simulink model "s_b4a4x32kf"  (R2018a)
settings: Solver=VariableStepDiscrete  StartTime=0.0  StopTime=1  RelTol=1e-3
undefined symbols (not defined in the file): fft_stages, n_bits_ants, n_bits_xengs
libraries: xbsIndex_r4 x22056, xbsReplacements_r4 x30, casper_library_misc x29, casper_library_scopes x15, xps_library x4
(part 125 of 227)

== system s_b4a4x32kf/sys0/xeng/auto_tap/dual_pol_cmac ==
  a1 : Inport
  a2 : Inport  Port=2
  acc_in : Inport  Port=3
  sync : Inport  Port=4
  valid_in : Inport  Port=5
  Concat : xbsIndex_r4/Concat  num_inputs=4  dbl_ovrd=off  block_type=concat
      settings: block_version=9.2.01
  Constant1 : xbsIndex_r4/Constant  const=0  gui_display_data_type=Fixed-point  arith_type=Unsigned  n_bits=1  bin_pt=0  preci_type=Single  exp_width=8  frac_width=24  explicit_period=on  period=1  equ=P=C  opselect=C  inp2=PCIN>>17  opr=+  inp1=P  carry=CIN  dbl_ovrd=off  block_type=constant
      settings: block_version=9.2.01
  Constant2 : xbsIndex_r4/Constant  const=0  gui_display_data_type=Fixed-point  arith_type=Unsigned  n_bits=1  bin_pt=0  preci_type=Single  exp_width=8  frac_width=24  explicit_period=on  period=1  equ=P=C  opselect=C  inp2=PCIN>>17  opr=+  inp1=P  carry=CIN  dbl_ovrd=off  block_type=constant
      settings: block_version=9.2.01
  Constant4 : xbsIndex_r4/Constant  const=0  gui_display_data_type=Fixed-point  arith_type=Unsigned  n_bits=1  bin_pt=0  preci_type=Single  exp_width=8  frac_width=24  explicit_period=on  period=1  equ=P=C  opselect=C  inp2=PCIN>>17  opr=+  inp1=P  carry=CIN  dbl_ovrd=off  block_type=constant
      settings: block_version=9.2.01
  Slice{,1,6,10} (4 alike) : xbsIndex_r4/Slice  nbits=2*n_bits  boolean_output=off  mode=Upper Bit Location + Width  bit1=0  base1=MSB of Input  bit0=0  base0=LSB of Input  dbl_ovrd=off  block_type=slice
      Slice settings: infoedit="Extracts a given range of bits from each input sample and presents it at the output.  The output type is ordinarily unsigned with binary point at zero, but can be Boolean when the slice is one bit wide.<P><P>Hardware notes: In hardware this block costs nothing."  block_version=9.2.01
      Slice1 settings: infoedit="Extracts a given range of bits from each input sample and presents it at the output.  The output type is ordinarily unsigned with binary point at zero, but can be Boolean when the slice is one bit wide.<P><P>Hardware notes: In hardware this block costs nothing."  block_version=9.2.01
      Slice10 settings: block_version=9.2.01
      Slice6 settings: infoedit="Extracts a given range of bits from each input sample and presents it at the output.  The output type is ordinarily unsigned with binary point at zero, but can be Boolean when the slice is one bit wide.<P><P>Hardware notes: In hardware this block costs nothing."  block_version=9.2.01
  Slice11 : xbsIndex_r4/Slice  nbits=2*n_bits_out  boolean_output=off  mode=Upper Bit Location + Width  bit1=-6*n_bits_out  base1=MSB of Input  bit0=0  base0=LSB of Input  dbl_ovrd=off  block_type=slice
      settings: infoedit="Extracts a given range of bits from each input sample and presents it at the output.  The output type is ordinarily unsigned with binary point at zero, but can be Boolean when the slice is one bit wide.<P><P>Hardware notes: In hardware this block costs nothing."  block_version=9.2.01
  Slice2 : xbsIndex_r4/Slice  nbits=2*n_bits_out  boolean_output=off  mode=Upper Bit Location + Width  bit1=0  base1=MSB of Input  bit0=0  base0=LSB of Input  dbl_ovrd=off  block_type=slice
      settings: infoedit="Extracts a given range of bits from each input sample and presents it at the output.  The output type is ordinarily unsigned with binary point at zero, but can be Boolean when the slice is one bit wide.<P><P>Hardware notes: In hardware this block costs nothing."  block_version=9.2.01
  Slice{3..4,7,9} (4 alike) : xbsIndex_r4/Slice  nbits=2*n_bits  boolean_output=off  mode=Upper Bit Location + Width  bit1=-2*n_bits  base1=MSB of Input  bit0=0  base0=LSB of Input  dbl_ovrd=off  block_type=slice
      Slice3 settings: infoedit="Extracts a given range of bits from each input sample and presents it at the output.  The output type is ordinarily unsigned with binary point at zero, but can be Boolean when the slice is one bit wide.<P><P>Hardware notes: In hardware this block costs nothing."  block_version=9.2.01
      Slice4 settings: infoedit="Extracts a given range of bits from each input sample and presents it at the output.  The output type is ordinarily unsigned with binary point at zero, but can be Boolean when the slice is one bit wide.<P><P>Hardware notes: In hardware this block costs nothing."  block_version=9.2.01
      Slice7 settings: infoedit="Extracts a given range of bits from each input sample and presents it at the output.  The output type is ordinarily unsigned with binary point at zero, but can be Boolean when the slice is one bit wide.<P><P>Hardware notes: In hardware this block costs nothing."  block_version=9.2.01
      Slice9 settings: block_version=9.2.01
  Slice5 : xbsIndex_r4/Slice  nbits=2*n_bits_out  boolean_output=off  mode=Upper Bit Location + Width  bit1=-2*n_bits_out  base1=MSB of Input  bit0=0  base0=LSB of Input  dbl_ovrd=off  block_type=slice
      settings: infoedit="Extracts a given range of bits from each input sample and presents it at the output.  The output type is ordinarily unsigned with binary point at zero, but can be Boolean when the slice is one bit wide.<P><P>Hardware notes: In hardware this block costs nothing."  block_version=9.2.01
  Slice8 : xbsIndex_r4/Slice  nbits=2*n_bits_out  boolean_output=off  mode=Upper Bit Location + Width  bit1=-4*n_bits_out  base1=MSB of Input  bit0=0  base0=LSB of Input  dbl_ovrd=off  block_type=slice
      settings: infoedit="Extracts a given range of bits from each input sample and presents it at the output.  The output type is ordinarily unsigned with binary point at zero, but can be Boolean when the slice is one bit wide.<P><P>Hardware notes: In hardware this block costs nothing."  block_version=9.2.01
  Terminator : Terminator
  Terminator1 : Terminator
  Terminator2 : Terminator
  cmac1 : Subsystem  Tag=cmac_delinked  mask(cmac){acc_len=256, n_bits_a=8, bin_pt_a=7, n_bits_b=8, bin_pt_b=7, quantization=Truncate, overflow=Wrap, mult_latency=4, add_latency=3, in_latency=0, conv_latency=0, multiplier_implementation=embedded multiplier core}
      mask prompts: acc_len "Number of Accumulations"; n_bits_a "Number of bits 'a'"; bin_pt_a "Binary point 'a'"; n_bits_b "Number of bits 'b'"; bin_pt_b "Binary point 'b'"; quantization "Quantisation"; mult_latency "Multiplier Latency"; add_latency "Adder Latency"; in_latency "Input Latency"; conv_latency "Convert Latency"; multiplier_implementation "Multiplier Implementation"
      mask help: A complex multiply-accumulate block. Full precision.
      mask init:
      | bit_growth = ceil(log2(acc_len));
      | n_bits_out = (n_bits_a + n_bits_b + 1 + bit_growth);
      | bin_pt_out=(bin_pt_a + bin_pt_b);
      | set_param(gcb,'LinkStatus','inactive');
      | set_param([gcb,'/cmult*'],'LinkStatus','inactive');
      | set_param([gcb,'/cmult*'],'multiplier_implementation',num2str(multiplier_implementation));
      | set_param([gcb,'/cmult*'],'mult_latency',num2str(mult_latency));
      | set_param([gcb,'/cmult*'],'conjugated','on');
      | set_param([gcb,'/cmult*'],'add_latency',num2str(add_latency));
      | set_param([gcb,'/cmult*'],'n_bits_ab',num2str(n_bits_out));
      | set_param([gcb,'/cmult*'],'n_bits_a',num2str(n_bits_a));
      | set_param([gcb,'/cmult*'],'n_bits_b',num2str(n_bits_b));
      | set_param([gcb,'/cmult*'],'bin_pt_a',num2str(bin_pt_a));
      | set_param([gcb,'/cmult*'],'bin_pt_b',num2str(bin_pt_b));
      | set_param([gcb,'/cmult*'],'bin_pt_ab',num2str(bin_pt_out));
      mask TypeOptions quantization: Truncate | Round  (unbiased: +/- Inf) | Round  (unbiased: Even Values)
      mask TypeOptions overflow: Wrap | Saturate | Flag as error
      mask TypeOptions multiplier_implementation: behavioral HDL | standard core | embedded multiplier core
  cmac2 : Subsystem  Tag=cmac_delinked  mask(cmac){acc_len=256, n_bits_a=8, bin_pt_a=7, n_bits_b=8, bin_pt_b=7, quantization=Truncate, overflow=Wrap, mult_latency=4, add_latency=3, in_latency=0, conv_latency=0, multiplier_implementation=embedded multiplier core}
      mask prompts: acc_len "Number of Accumulations"; n_bits_a "Number of bits 'a'"; bin_pt_a "Binary point 'a'"; n_bits_b "Number of bits 'b'"; bin_pt_b "Binary point 'b'"; quantization "Quantisation"; mult_latency "Multiplier Latency"; add_latency "Adder Latency"; in_latency "Input Latency"; conv_latency "Convert Latency"; multiplier_implementation "Multiplier Implementation"
      mask help: A complex multiply-accumulate block. Full precision.
      mask init: same as s_b4a4x32kf/sys0/xeng/auto_tap/dual_pol_cmac/cmac1
      mask TypeOptions quantization: Truncate | Round  (unbiased: +/- Inf) | Round  (unbiased: Even Values)
      mask TypeOptions overflow: Wrap | Saturate | Flag as error
      mask TypeOptions multiplier_implementation: behavioral HDL | standard core | embedded multiplier core
  cmac3 : Subsystem  Tag=cmac_delinked  mask(cmac){acc_len=256, n_bits_a=8, bin_pt_a=7, n_bits_b=8, bin_pt_b=7, quantization=Truncate, overflow=Wrap, mult_latency=4, add_latency=3, in_latency=0, conv_latency=0, multiplier_implementation=embedded multiplier core}
      mask prompts: acc_len "Number of Accumulations"; n_bits_a "Number of bits 'a'"; bin_pt_a "Binary point 'a'"; n_bits_b "Number of bits 'b'"; bin_pt_b "Binary point 'b'"; quantization "Quantisation"; mult_latency "Multiplier Latency"; add_latency "Adder Latency"; in_latency "Input Latency"; conv_latency "Convert Latency"; multiplier_implementation "Multiplier Implementation"
      mask help: A complex multiply-accumulate block. Full precision.
      mask init: same as s_b4a4x32kf/sys0/xeng/auto_tap/dual_pol_cmac/cmac1
      mask TypeOptions quantization: Truncate | Round  (unbiased: +/- Inf) | Round  (unbiased: Even Values)
      mask TypeOptions overflow: Wrap | Saturate | Flag as error
      mask TypeOptions multiplier_implementation: behavioral HDL | standard core | embedded multiplier core
  cmac4 : Subsystem  Tag=cmac_delinked  mask(cmac){acc_len=256, n_bits_a=8, bin_pt_a=7, n_bits_b=8, bin_pt_b=7, quantization=Truncate, overflow=Wrap, mult_latency=4, add_latency=3, in_latency=0, conv_latency=0, multiplier_implementation=embedded multiplier core}
      mask prompts: acc_len "Number of Accumulations"; n_bits_a "Number of bits 'a'"; bin_pt_a "Binary point 'a'"; n_bits_b "Number of bits 'b'"; bin_pt_b "Binary point 'b'"; quantization "Quantisation"; mult_latency "Multiplier Latency"; add_latency "Adder Latency"; in_latency "Input Latency"; conv_latency "Convert Latency"; multiplier_implementation "Multiplier Implementation"
      mask help: A complex multiply-accumulate block. Full precision.
      mask init: same as s_b4a4x32kf/sys0/xeng/auto_tap/dual_pol_cmac/cmac1
      mask TypeOptions quantization: Truncate | Round  (unbiased: +/- Inf) | Round  (unbiased: Even Values)
      mask TypeOptions overflow: Wrap | Saturate | Flag as error
      mask TypeOptions multiplier_implementation: behavioral HDL | standard core | embedded multiplier core
  acc_out : Outport
  valid_out : Outport  Port=2
  wires:
  acc_in/1 -> Slice2/1, Slice5/1, Slice8/1, Slice11/1
  a2/1 -> Slice10/1, Slice7/1, Slice4/1, Slice1/1
  a1/1 -> Slice9/1, Slice6/1, Slice3/1, Slice/1
  cmac4/1(acc_out) -> Concat/4
  cmac3/1(acc_out) -> Concat/3
  cmac2/1(acc_out) -> Concat/2
  cmac1/1(acc_out) -> Concat/1
  cmac4/2(valid_out) -> valid_out/1
  cmac3/2(valid_out) -> Terminator2/1
  cmac2/2(valid_out) -> Terminator1/1
  sync/1 -> cmac4/4(sync), cmac3/4(sync), cmac2/4(sync), cmac1/4(sync)
  Slice11/1 -> cmac4/3(acc_in)
  Slice10/1 -> cmac4/2(c+di)
  Slice9/1 -> cmac4/1(a+bi)
  Constant4/1 -> cmac3/5(valid_in)
  Slice8/1 -> cmac3/3(acc_in)
  Slice7/1 -> cmac3/2(c+di)
  Slice6/1 -> cmac3/1(a+bi)
  Constant1/1 -> cmac2/5(valid_in)
  cmac1/2(valid_out) -> Terminator/1
  valid_in/1 -> cmac4/5(valid_in)
  Concat/1 -> acc_out/1
  Slice5/1 -> cmac2/3(acc_in)
  Slice4/1 -> cmac2/2(c+di)
  Slice3/1 -> cmac2/1(a+bi)
  Slice2/1 -> cmac1/3(acc_in)
  Slice1/1 -> cmac1/2(c+di)
  Slice/1 -> cmac1/1(a+bi)
  Constant2/1 -> cmac1/5(valid_in)

== system s_b4a4x32kf/sys0/xeng/auto_tap/sync_delay ==
  In : Inport
  Constant : xbsIndex_r4/Constant  const=1  gui_display_data_type=Fixed-point  arith_type=Unsigned  n_bits=BitWidth  bin_pt=0  preci_type=Single  exp_width=8  frac_width=24  explicit_period=on  period=1  equ=P=C  opselect=C  inp2=PCIN>>17  opr=+  inp1=P  carry=CIN  dbl_ovrd=off  block_type=constant
      settings: block_version=9.1.01
  Constant1 : xbsIndex_r4/Constant  const=0  gui_display_data_type=Fixed-point  arith_type=Unsigned  n_bits=BitWidth  bin_pt=0  preci_type=Single  exp_width=8  frac_width=24  explicit_period=on  period=1  equ=P=C  opselect=C  inp2=PCIN>>17  opr=+  inp1=P  carry=CIN  dbl_ovrd=off  block_type=constant
      settings: block_version=9.1.01
  Constant2 : xbsIndex_r4/Constant  const=DelayLen  gui_display_data_type=Fixed-point  arith_type=Unsigned  n_bits=BitWidth  bin_pt=0  preci_type=Single  exp_width=8  frac_width=24  explicit_period=on  period=1  equ=P=C  opselect=C  inp2=PCIN>>17  opr=+  inp1=P  carry=CIN  dbl_ovrd=off  block_type=constant
      settings: block_version=9.1.01
  Constant3 : xbsIndex_r4/Constant  const=UseCounter  gui_display_data_type=Fixed-point  arith_type=Unsigned  n_bits=1  bin_pt=0  preci_type=Single  exp_width=8  frac_width=24  explicit_period=on  period=1  equ=P=C  opselect=C  inp2=PCIN>>17  opr=+  inp1=P  carry=CIN  dbl_ovrd=off  block_type=constant
      settings: block_version=9.1.01
  Counter : xbsIndex_r4/Counter  cnt_type=Free Running  cnt_to=Inf  operation=Down  start_count=0  cnt_by_val=1  arith_type=Unsigned  n_bits=BitWidth  bin_pt=0  load_pin=on  rst=off  en=on  explicit_period=on  period=1  use_behavioral_HDL=off  implementation=Fabric  use_rpm=on  dbl_ovrd=off  block_type=counter
      settings: xl_area=[0, 0, 0, 0, 0, 0, 0]  block_version=9.1.01
  Logical : xbsIndex_r4/Logical  logical_function=OR  inputs=2  en=off  latency=0  precision=Full  arith_type=Unsigned  n_bits=8  bin_pt=2  align_bp=on  dbl_ovrd=off  block_type=logical
      settings: xl_area=[0, 0, 0, 0, 0, 0, 0]  block_version=9.1.01
  Mux : xbsIndex_r4/Mux  inputs=2  en=off  latency=0  precision=Full  arith_type="Signed  (2's comp)"  n_bits=8  bin_pt=2  quantization=Truncate  overflow=Wrap  dbl_ovrd=off  block_type=mux
      settings: xl_area=[0, 0, 0, 0, 0, 0, 0]  block_version=9.1.01
  Relational : xbsIndex_r4/Relational  mode=a=b  op_type=Bool  en=off  latency=0  dbl_ovrd=off  block_type=relational
      settings: xl_area=[0, 0, 0, 0, 0, 0, 0]  block_version=9.1.01
  Relational1 : xbsIndex_r4/Relational  mode=a!=b  op_type=Bool  en=off  latency=0  dbl_ovrd=off  block_type=relational
      settings: xl_area=[0, 0, 0, 0, 0, 0, 0]  block_version=9.1.01
  warn period Logical0 : xbsReplacements_r4/Warning  period=1
  warn period Relational10 : xbsReplacements_r4/Warning  period=1
  Out : Outport
  wires:
  Mux/1 -> Out/1
  Constant3/1 -> Mux/1
  Relational/1 -> Mux/3
  Relational1/1 -> Logical/2
  Logical/1 -> Counter/3
  In/1 -> Mux/2, Logical/1, Counter/1
  Constant2/1 -> Counter/2
  Constant/1 -> Relational/1
  Constant1/1 -> Relational1/2
  Counter/1 -> Relational/2, Relational1/1

== system s_b4a4x32kf/sys0/xeng/baseline_tap1/delay ==
  din : Inport
  constant : xbsIndex_r4/Constant  const=1  gui_display_data_type=Fixed-point  arith_type=Boolean  n_bits=16  bin_pt=14  preci_type=Single  exp_width=8  frac_width=24  explicit_period=on  period=1  equ=P=C  opselect=C  inp2=PCIN>>17  opr=+  inp1=P  carry=CIN  dbl_ovrd=off  block_type=constant
  counter : xbsIndex_r4/Counter  cnt_type=Count Limited  cnt_to=DelayLen - bram_latency - 1  operation=Up  start_count=0  cnt_by_val=1  arith_type=Unsigned  n_bits=8  bin_pt=0  load_pin=off  rst=off  en=off  explicit_period=on  period=1  use_behavioral_HDL=on  implementation=Fabric  use_rpm=off  dbl_ovrd=off  block_type=counter
  ram : xbsIndex_r4/Single Port RAM  depth=256  initVector=0  distributed_mem=Block RAM  write_mode=Read Before Write  rst=off  init_reg=0  en=off  latency=bram_latency  optimize=Area  dbl_ovrd=off  block_type=spram
  dout : Outport
  wires:
  counter/1 -> ram/1
  din/1 -> ram/2
  constant/1 -> ram/3
  ram/1 -> dout/1

== system s_b4a4x32kf/sys0/xeng/baseline_tap1/dual_pol_cmac ==
  a1 : Inport
  a2 : Inport  Port=2
  acc_in : Inport  Port=3
  sync : Inport  Port=4
  valid_in : Inport  Port=5
  Concat : xbsIndex_r4/Concat  num_inputs=4  dbl_ovrd=off  block_type=concat
      settings: block_version=9.2.01
  Constant1 : xbsIndex_r4/Constant  const=0  gui_display_data_type=Fixed-point  arith_type=Unsigned  n_bits=1  bin_pt=0  preci_type=Single  exp_width=8  frac_width=24  explicit_period=on  period=1  equ=P=C  opselect=C  inp2=PCIN>>17  opr=+  inp1=P  carry=CIN  dbl_ovrd=off  block_type=constant
      settings: block_version=9.2.01
  Constant2 : xbsIndex_r4/Constant  const=0  gui_display_data_type=Fixed-point  arith_type=Unsigned  n_bits=1  bin_pt=0  preci_type=Single  exp_width=8  frac_width=24  explicit_period=on  period=1  equ=P=C  opselect=C  inp2=PCIN>>17  opr=+  inp1=P  carry=CIN  dbl_ovrd=off  block_type=constant
      settings: block_version=9.2.01
  Constant4 : xbsIndex_r4/Constant  const=0  gui_display_data_type=Fixed-point  arith_type=Unsigned  n_bits=1  bin_pt=0  preci_type=Single  exp_width=8  frac_width=24  explicit_period=on  period=1  equ=P=C  opselect=C  inp2=PCIN>>17  opr=+  inp1=P  carry=CIN  dbl_ovrd=off  block_type=constant
      settings: block_version=9.2.01
  Slice{,1,6,10} (4 alike) : xbsIndex_r4/Slice  nbits=2*n_bits  boolean_output=off  mode=Upper Bit Location + Width  bit1=0  base1=MSB of Input  bit0=0  base0=LSB of Input  dbl_ovrd=off  block_type=slice
      Slice settings: infoedit="Extracts a given range of bits from each input sample and presents it at the output.  The output type is ordinarily unsigned with binary point at zero, but can be Boolean when the slice is one bit wide.<P><P>Hardware notes: In hardware this block costs nothing."  block_version=9.2.01
      Slice1 settings: infoedit="Extracts a given range of bits from each input sample and presents it at the output.  The output type is ordinarily unsigned with binary point at zero, but can be Boolean when the slice is one bit wide.<P><P>Hardware notes: In hardware this block costs nothing."  block_version=9.2.01
      Slice10 settings: block_version=9.2.01
      Slice6 settings: infoedit="Extracts a given range of bits from each input sample and presents it at the output.  The output type is ordinarily unsigned with binary point at zero, but can be Boolean when the slice is one bit wide.<P><P>Hardware notes: In hardware this block costs nothing."  block_version=9.2.01
  Slice11 : xbsIndex_r4/Slice  nbits=2*n_bits_out  boolean_output=off  mode=Upper Bit Location + Width  bit1=-6*n_bits_out  base1=MSB of Input  bit0=0  base0=LSB of Input  dbl_ovrd=off  block_type=slice
      settings: infoedit="Extracts a given range of bits from each input sample and presents it at the output.  The output type is ordinarily unsigned with binary point at zero, but can be Boolean when the slice is one bit wide.<P><P>Hardware notes: In hardware this block costs nothing."  block_version=9.2.01
  Slice2 : xbsIndex_r4/Slice  nbits=2*n_bits_out  boolean_output=off  mode=Upper Bit Location + Width  bit1=0  base1=MSB of Input  bit0=0  base0=LSB of Input  dbl_ovrd=off  block_type=slice
      settings: infoedit="Extracts a given range of bits from each input sample and presents it at the output.  The output type is ordinarily unsigned with binary point at zero, but can be Boolean when the slice is one bit wide.<P><P>Hardware notes: In hardware this block costs nothing."  block_version=9.2.01
  Slice{3..4,7,9} (4 alike) : xbsIndex_r4/Slice  nbits=2*n_bits  boolean_output=off  mode=Upper Bit Location + Width  bit1=-2*n_bits  base1=MSB of Input  bit0=0  base0=LSB of Input  dbl_ovrd=off  block_type=slice
      Slice3 settings: infoedit="Extracts a given range of bits from each input sample and presents it at the output.  The output type is ordinarily unsigned with binary point at zero, but can be Boolean when the slice is one bit wide.<P><P>Hardware notes: In hardware this block costs nothing."  block_version=9.2.01
      Slice4 settings: infoedit="Extracts a given range of bits from each input sample and presents it at the output.  The output type is ordinarily unsigned with binary point at zero, but can be Boolean when the slice is one bit wide.<P><P>Hardware notes: In hardware this block costs nothing."  block_version=9.2.01
      Slice7 settings: infoedit="Extracts a given range of bits from each input sample and presents it at the output.  The output type is ordinarily unsigned with binary point at zero, but can be Boolean when the slice is one bit wide.<P><P>Hardware notes: In hardware this block costs nothing."  block_version=9.2.01
      Slice9 settings: block_version=9.2.01
  Slice5 : xbsIndex_r4/Slice  nbits=2*n_bits_out  boolean_output=off  mode=Upper Bit Location + Width  bit1=-2*n_bits_out  base1=MSB of Input  bit0=0  base0=LSB of Input  dbl_ovrd=off  block_type=slice
      settings: infoedit="Extracts a given range of bits from each input sample and presents it at the output.  The output type is ordinarily unsigned with binary point at zero, but can be Boolean when the slice is one bit wide.<P><P>Hardware notes: In hardware this block costs nothing."  block_version=9.2.01
  Slice8 : xbsIndex_r4/Slice  nbits=2*n_bits_out  boolean_output=off  mode=Upper Bit Location + Width  bit1=-4*n_bits_out  base1=MSB of Input  bit0=0  base0=LSB of Input  dbl_ovrd=off  block_type=slice
      settings: infoedit="Extracts a given range of bits from each input sample and presents it at the output.  The output type is ordinarily unsigned with binary point at zero, but can be Boolean when the slice is one bit wide.<P><P>Hardware notes: In hardware this block costs nothing."  block_version=9.2.01
  Terminator : Terminator
  Terminator1 : Terminator
  Terminator2 : Terminator
  cmac1 : Subsystem  Tag=cmac_delinked  mask(cmac){acc_len=256, n_bits_a=8, bin_pt_a=7, n_bits_b=8, bin_pt_b=7, quantization=Truncate, overflow=Wrap, mult_latency=4, add_latency=3, in_latency=0, conv_latency=0, multiplier_implementation=embedded multiplier core}
      mask prompts: acc_len "Number of Accumulations"; n_bits_a "Number of bits 'a'"; bin_pt_a "Binary point 'a'"; n_bits_b "Number of bits 'b'"; bin_pt_b "Binary point 'b'"; quantization "Quantisation"; mult_latency "Multiplier Latency"; add_latency "Adder Latency"; in_latency "Input Latency"; conv_latency "Convert Latency"; multiplier_implementation "Multiplier Implementation"
      mask help: A complex multiply-accumulate block. Full precision.
      mask init: same as s_b4a4x32kf/sys0/xeng/auto_tap/dual_pol_cmac/cmac1
      mask TypeOptions quantization: Truncate | Round  (unbiased: +/- Inf) | Round  (unbiased: Even Values)
      mask TypeOptions overflow: Wrap | Saturate | Flag as error
      mask TypeOptions multiplier_implementation: behavioral HDL | standard core | embedded multiplier core
  cmac2 : Subsystem  Tag=cmac_delinked  mask(cmac){acc_len=256, n_bits_a=8, bin_pt_a=7, n_bits_b=8, bin_pt_b=7, quantization=Truncate, overflow=Wrap, mult_latency=4, add_latency=3, in_latency=0, conv_latency=0, multiplier_implementation=embedded multiplier core}
      mask prompts: acc_len "Number of Accumulations"; n_bits_a "Number of bits 'a'"; bin_pt_a "Binary point 'a'"; n_bits_b "Number of bits 'b'"; bin_pt_b "Binary point 'b'"; quantization "Quantisation"; mult_latency "Multiplier Latency"; add_latency "Adder Latency"; in_latency "Input Latency"; conv_latency "Convert Latency"; multiplier_implementation "Multiplier Implementation"
      mask help: A complex multiply-accumulate block. Full precision.
      mask init: same as s_b4a4x32kf/sys0/xeng/auto_tap/dual_pol_cmac/cmac1
      mask TypeOptions quantization: Truncate | Round  (unbiased: +/- Inf) | Round  (unbiased: Even Values)
      mask TypeOptions overflow: Wrap | Saturate | Flag as error
      mask TypeOptions multiplier_implementation: behavioral HDL | standard core | embedded multiplier core
  cmac3 : Subsystem  Tag=cmac_delinked  mask(cmac){acc_len=256, n_bits_a=8, bin_pt_a=7, n_bits_b=8, bin_pt_b=7, quantization=Truncate, overflow=Wrap, mult_latency=4, add_latency=3, in_latency=0, conv_latency=0, multiplier_implementation=embedded multiplier core}
      mask prompts: acc_len "Number of Accumulations"; n_bits_a "Number of bits 'a'"; bin_pt_a "Binary point 'a'"; n_bits_b "Number of bits 'b'"; bin_pt_b "Binary point 'b'"; quantization "Quantisation"; mult_latency "Multiplier Latency"; add_latency "Adder Latency"; in_latency "Input Latency"; conv_latency "Convert Latency"; multiplier_implementation "Multiplier Implementation"
      mask help: A complex multiply-accumulate block. Full precision.
      mask init: same as s_b4a4x32kf/sys0/xeng/auto_tap/dual_pol_cmac/cmac1
      mask TypeOptions quantization: Truncate | Round  (unbiased: +/- Inf) | Round  (unbiased: Even Values)
      mask TypeOptions overflow: Wrap | Saturate | Flag as error
      mask TypeOptions multiplier_implementation: behavioral HDL | standard core | embedded multiplier core
  cmac4 : Subsystem  Tag=cmac_delinked  mask(cmac){acc_len=256, n_bits_a=8, bin_pt_a=7, n_bits_b=8, bin_pt_b=7, quantization=Truncate, overflow=Wrap, mult_latency=4, add_latency=3, in_latency=0, conv_latency=0, multiplier_implementation=embedded multiplier core}
      mask prompts: acc_len "Number of Accumulations"; n_bits_a "Number of bits 'a'"; bin_pt_a "Binary point 'a'"; n_bits_b "Number of bits 'b'"; bin_pt_b "Binary point 'b'"; quantization "Quantisation"; mult_latency "Multiplier Latency"; add_latency "Adder Latency"; in_latency "Input Latency"; conv_latency "Convert Latency"; multiplier_implementation "Multiplier Implementation"
      mask help: A complex multiply-accumulate block. Full precision.
      mask init: same as s_b4a4x32kf/sys0/xeng/auto_tap/dual_pol_cmac/cmac1
      mask TypeOptions quantization: Truncate | Round  (unbiased: +/- Inf) | Round  (unbiased: Even Values)
      mask TypeOptions overflow: Wrap | Saturate | Flag as error
      mask TypeOptions multiplier_implementation: behavioral HDL | standard core | embedded multiplier core
  acc_out : Outport
  valid_out : Outport  Port=2
  wires:
  acc_in/1 -> Slice2/1, Slice5/1, Slice8/1, Slice11/1
  a2/1 -> Slice10/1, Slice7/1, Slice4/1, Slice1/1
  a1/1 -> Slice9/1, Slice6/1, Slice3/1, Slice/1
  cmac4/1(acc_out) -> Concat/4
  cmac3/1(acc_out) -> Concat/3
  cmac2/1(acc_out) -> Concat/2
  cmac1/1(acc_out) -> Concat/1
  cmac4/2(valid_out) -> valid_out/1
  cmac3/2(valid_out) -> Terminator2/1
  cmac2/2(valid_out) -> Terminator1/1
  sync/1 -> cmac4/4(sync), cmac3/4(sync), cmac2/4(sync), cmac1/4(sync)
  Slice11/1 -> cmac4/3(acc_in)
  Slice10/1 -> cmac4/2(c+di)
  Slice9/1 -> cmac4/1(a+bi)
  Constant4/1 -> cmac3/5(valid_in)
  Slice8/1 -> cmac3/3(acc_in)
  Slice7/1 -> cmac3/2(c+di)
  Slice6/1 -> cmac3/1(a+bi)
  Constant1/1 -> cmac2/5(valid_in)
  cmac1/2(valid_out) -> Terminator/1
  valid_in/1 -> cmac4/5(valid_in)
  Concat/1 -> acc_out/1
  Slice5/1 -> cmac2/3(acc_in)
  Slice4/1 -> cmac2/2(c+di)
  Slice3/1 -> cmac2/1(a+bi)
  Slice2/1 -> cmac1/3(acc_in)
  Slice1/1 -> cmac1/2(c+di)
  Slice/1 -> cmac1/1(a+bi)
  Constant2/1 -> cmac1/5(valid_in)

== system s_b4a4x32kf/sys0/xeng/baseline_tap2/delay ==
  din : Inport
  constant : xbsIndex_r4/Constant  const=1  gui_display_data_type=Fixed-point  arith_type=Boolean  n_bits=16  bin_pt=14  preci_type=Single  exp_width=8  frac_width=24  explicit_period=on  period=1  equ=P=C  opselect=C  inp2=PCIN>>17  opr=+  inp1=P  carry=CIN  dbl_ovrd=off  block_type=constant
  counter : xbsIndex_r4/Counter  cnt_type=Count Limited  cnt_to=DelayLen - bram_latency - 1  operation=Up  start_count=0  cnt_by_val=1  arith_type=Unsigned  n_bits=8  bin_pt=0  load_pin=off  rst=off  en=off  explicit_period=on  period=1  use_behavioral_HDL=on  implementation=Fabric  use_rpm=off  dbl_ovrd=off  block_type=counter
  ram : xbsIndex_r4/Single Port RAM  depth=256  initVector=0  distributed_mem=Block RAM  write_mode=Read Before Write  rst=off  init_reg=0  en=off  latency=bram_latency  optimize=Area  dbl_ovrd=off  block_type=spram
  dout : Outport
  wires:
  counter/1 -> ram/1
  din/1 -> ram/2
  constant/1 -> ram/3
  ram/1 -> dout/1

== system s_b4a4x32kf/sys0/xeng/baseline_tap2/dual_pol_cmac ==
  a1 : Inport
  a2 : Inport  Port=2
  acc_in : Inport  Port=3
  sync : Inport  Port=4
  valid_in : Inport  Port=5
  Concat : xbsIndex_r4/Concat  num_inputs=4  dbl_ovrd=off  block_type=concat
      settings: block_version=9.2.01
  Constant1 : xbsIndex_r4/Constant  const=0  gui_display_data_type=Fixed-point  arith_type=Unsigned  n_bits=1  bin_pt=0  preci_type=Single  exp_width=8  frac_width=24  explicit_period=on  period=1  equ=P=C  opselect=C  inp2=PCIN>>17  opr=+  inp1=P  carry=CIN  dbl_ovrd=off  block_type=constant
      settings: block_version=9.2.01
  Constant2 : xbsIndex_r4/Constant  const=0  gui_display_data_type=Fixed-point  arith_type=Unsigned  n_bits=1  bin_pt=0  preci_type=Single  exp_width=8  frac_width=24  explicit_period=on  period=1  equ=P=C  opselect=C  inp2=PCIN>>17  opr=+  inp1=P  carry=CIN  dbl_ovrd=off  block_type=constant
      settings: block_version=9.2.01
  Constant4 : xbsIndex_r4/Constant  const=0  gui_display_data_type=Fixed-point  arith_type=Unsigned  n_bits=1  bin_pt=0  preci_type=Single  exp_width=8  frac_width=24  explicit_period=on  period=1  equ=P=C  opselect=C  inp2=PCIN>>17  opr=+  inp1=P  carry=CIN  dbl_ovrd=off  block_type=constant
      settings: block_version=9.2.01
  Slice{,1,6,10} (4 alike) : xbsIndex_r4/Slice  nbits=2*n_bits  boolean_output=off  mode=Upper Bit Location + Width  bit1=0  base1=MSB of Input  bit0=0  base0=LSB of Input  dbl_ovrd=off  block_type=slice
      Slice settings: infoedit="Extracts a given range of bits from each input sample and presents it at the output.  The output type is ordinarily unsigned with binary point at zero, but can be Boolean when the slice is one bit wide.<P><P>Hardware notes: In hardware this block costs nothing."  block_version=9.2.01
      Slice1 settings: infoedit="Extracts a given range of bits from each input sample and presents it at the output.  The output type is ordinarily unsigned with binary point at zero, but can be Boolean when the slice is one bit wide.<P><P>Hardware notes: In hardware this block costs nothing."  block_version=9.2.01
      Slice10 settings: block_version=9.2.01
      Slice6 settings: infoedit="Extracts a given range of bits from each input sample and presents it at the output.  The output type is ordinarily unsigned with binary point at zero, but can be Boolean when the slice is one bit wide.<P><P>Hardware notes: In hardware this block costs nothing."  block_version=9.2.01
  Slice11 : xbsIndex_r4/Slice  nbits=2*n_bits_out  boolean_output=off  mode=Upper Bit Location + Width  bit1=-6*n_bits_out  base1=MSB of Input  bit0=0  base0=LSB of Input  dbl_ovrd=off  block_type=slice
      settings: infoedit="Extracts a given range of bits from each input sample and presents it at the output.  The output type is ordinarily unsigned with binary point at zero, but can be Boolean when the slice is one bit wide.<P><P>Hardware notes: In hardware this block costs nothing."  block_version=9.2.01
  Slice2 : xbsIndex_r4/Slice  nbits=2*n_bits_out  boolean_output=off  mode=Upper Bit Location + Width  bit1=0  base1=MSB of Input  bit0=0  base0=LSB of Input  dbl_ovrd=off  block_type=slice
      settings: infoedit="Extracts a given range of bits from each input sample and presents it at the output.  The output type is ordinarily unsigned with binary point at zero, but can be Boolean when the slice is one bit wide.<P><P>Hardware notes: In hardware this block costs nothing."  block_version=9.2.01
  Slice{3..4,7,9} (4 alike) : xbsIndex_r4/Slice  nbits=2*n_bits  boolean_output=off  mode=Upper Bit Location + Width  bit1=-2*n_bits  base1=MSB of Input  bit0=0  base0=LSB of Input  dbl_ovrd=off  block_type=slice
      Slice3 settings: infoedit="Extracts a given range of bits from each input sample and presents it at the output.  The output type is ordinarily unsigned with binary point at zero, but can be Boolean when the slice is one bit wide.<P><P>Hardware notes: In hardware this block costs nothing."  block_version=9.2.01
      Slice4 settings: infoedit="Extracts a given range of bits from each input sample and presents it at the output.  The output type is ordinarily unsigned with binary point at zero, but can be Boolean when the slice is one bit wide.<P><P>Hardware notes: In hardware this block costs nothing."  block_version=9.2.01
      Slice7 settings: infoedit="Extracts a given range of bits from each input sample and presents it at the output.  The output type is ordinarily unsigned with binary point at zero, but can be Boolean when the slice is one bit wide.<P><P>Hardware notes: In hardware this block costs nothing."  block_version=9.2.01
      Slice9 settings: block_version=9.2.01
  Slice5 : xbsIndex_r4/Slice  nbits=2*n_bits_out  boolean_output=off  mode=Upper Bit Location + Width  bit1=-2*n_bits_out  base1=MSB of Input  bit0=0  base0=LSB of Input  dbl_ovrd=off  block_type=slice
      settings: infoedit="Extracts a given range of bits from each input sample and presents it at the output.  The output type is ordinarily unsigned with binary point at zero, but can be Boolean when the slice is one bit wide.<P><P>Hardware notes: In hardware this block costs nothing."  block_version=9.2.01
  Slice8 : xbsIndex_r4/Slice  nbits=2*n_bits_out  boolean_output=off  mode=Upper Bit Location + Width  bit1=-4*n_bits_out  base1=MSB of Input  bit0=0  base0=LSB of Input  dbl_ovrd=off  block_type=slice
      settings: infoedit="Extracts a given range of bits from each input sample and presents it at the output.  The output type is ordinarily unsigned with binary point at zero, but can be Boolean when the slice is one bit wide.<P><P>Hardware notes: In hardware this block costs nothing."  block_version=9.2.01
  Terminator : Terminator
  Terminator1 : Terminator
  Terminator2 : Terminator
  cmac1 : Subsystem  Tag=cmac_delinked  mask(cmac){acc_len=256, n_bits_a=8, bin_pt_a=7, n_bits_b=8, bin_pt_b=7, quantization=Truncate, overflow=Wrap, mult_latency=4, add_latency=3, in_latency=0, conv_latency=0, multiplier_implementation=embedded multiplier core}
      mask prompts: acc_len "Number of Accumulations"; n_bits_a "Number of bits 'a'"; bin_pt_a "Binary point 'a'"; n_bits_b "Number of bits 'b'"; bin_pt_b "Binary point 'b'"; quantization "Quantisation"; mult_latency "Multiplier Latency"; add_latency "Adder Latency"; in_latency "Input Latency"; conv_latency "Convert Latency"; multiplier_implementation "Multiplier Implementation"
      mask help: A complex multiply-accumulate block. Full precision.
      mask init: same as s_b4a4x32kf/sys0/xeng/auto_tap/dual_pol_cmac/cmac1
      mask TypeOptions quantization: Truncate | Round  (unbiased: +/- Inf) | Round  (unbiased: Even Values)
      mask TypeOptions overflow: Wrap | Saturate | Flag as error
      mask TypeOptions multiplier_implementation: behavioral HDL | standard core | embedded multiplier core
  cmac2 : Subsystem  Tag=cmac_delinked  mask(cmac){acc_len=256, n_bits_a=8, bin_pt_a=7, n_bits_b=8, bin_pt_b=7, quantization=Truncate, overflow=Wrap, mult_latency=4, add_latency=3, in_latency=0, conv_latency=0, multiplier_implementation=embedded multiplier core}
      mask prompts: acc_len "Number of Accumulations"; n_bits_a "Number of bits 'a'"; bin_pt_a "Binary point 'a'"; n_bits_b "Number of bits 'b'"; bin_pt_b "Binary point 'b'"; quantization "Quantisation"; mult_latency "Multiplier Latency"; add_latency "Adder Latency"; in_latency "Input Latency"; conv_latency "Convert Latency"; multiplier_implementation "Multiplier Implementation"
      mask help: A complex multiply-accumulate block. Full precision.
      mask init: same as s_b4a4x32kf/sys0/xeng/auto_tap/dual_pol_cmac/cmac1
      mask TypeOptions quantization: Truncate | Round  (unbiased: +/- Inf) | Round  (unbiased: Even Values)
      mask TypeOptions overflow: Wrap | Saturate | Flag as error
      mask TypeOptions multiplier_implementation: behavioral HDL | standard core | embedded multiplier core
  cmac3 : Subsystem  Tag=cmac_delinked  mask(cmac){acc_len=256, n_bits_a=8, bin_pt_a=7, n_bits_b=8, bin_pt_b=7, quantization=Truncate, overflow=Wrap, mult_latency=4, add_latency=3, in_latency=0, conv_latency=0, multiplier_implementation=embedded multiplier core}
      mask prompts: acc_len "Number of Accumulations"; n_bits_a "Number of bits 'a'"; bin_pt_a "Binary point 'a'"; n_bits_b "Number of bits 'b'"; bin_pt_b "Binary point 'b'"; quantization "Quantisation"; mult_latency "Multiplier Latency"; add_latency "Adder Latency"; in_latency "Input Latency"; conv_latency "Convert Latency"; multiplier_implementation "Multiplier Implementation"
      mask help: A complex multiply-accumulate block. Full precision.
      mask init: same as s_b4a4x32kf/sys0/xeng/auto_tap/dual_pol_cmac/cmac1
      mask TypeOptions quantization: Truncate | Round  (unbiased: +/- Inf) | Round  (unbiased: Even Values)
      mask TypeOptions overflow: Wrap | Saturate | Flag as error
      mask TypeOptions multiplier_implementation: behavioral HDL | standard core | embedded multiplier core
  cmac4 : Subsystem  Tag=cmac_delinked  mask(cmac){acc_len=256, n_bits_a=8, bin_pt_a=7, n_bits_b=8, bin_pt_b=7, quantization=Truncate, overflow=Wrap, mult_latency=4, add_latency=3, in_latency=0, conv_latency=0, multiplier_implementation=embedded multiplier core}
      mask prompts: acc_len "Number of Accumulations"; n_bits_a "Number of bits 'a'"; bin_pt_a "Binary point 'a'"; n_bits_b "Number of bits 'b'"; bin_pt_b "Binary point 'b'"; quantization "Quantisation"; mult_latency "Multiplier Latency"; add_latency "Adder Latency"; in_latency "Input Latency"; conv_latency "Convert Latency"; multiplier_implementation "Multiplier Implementation"
      mask help: A complex multiply-accumulate block. Full precision.
      mask init: same as s_b4a4x32kf/sys0/xeng/auto_tap/dual_pol_cmac/cmac1
      mask TypeOptions quantization: Truncate | Round  (unbiased: +/- Inf) | Round  (unbiased: Even Values)
      mask TypeOptions overflow: Wrap | Saturate | Flag as error
      mask TypeOptions multiplier_implementation: behavioral HDL | standard core | embedded multiplier core
  acc_out : Outport
  valid_out : Outport  Port=2
  wires:
  acc_in/1 -> Slice2/1, Slice5/1, Slice8/1, Slice11/1
  a2/1 -> Slice10/1, Slice7/1, Slice4/1, Slice1/1
  a1/1 -> Slice9/1, Slice6/1, Slice3/1, Slice/1
  cmac4/1(acc_out) -> Concat/4
  cmac3/1(acc_out) -> Concat/3
  cmac2/1(acc_out) -> Concat/2
  cmac1/1(acc_out) -> Concat/1
  cmac4/2(valid_out) -> valid_out/1
  cmac3/2(valid_out) -> Terminator2/1
  cmac2/2(valid_out) -> Terminator1/1
  sync/1 -> cmac4/4(sync), cmac3/4(sync), cmac2/4(sync), cmac1/4(sync)
  Slice11/1 -> cmac4/3(acc_in)
  Slice10/1 -> cmac4/2(c+di)
  Slice9/1 -> cmac4/1(a+bi)
  Constant4/1 -> cmac3/5(valid_in)
  Slice8/1 -> cmac3/3(acc_in)
  Slice7/1 -> cmac3/2(c+di)
  Slice6/1 -> cmac3/1(a+bi)
  Constant1/1 -> cmac2/5(valid_in)
  cmac1/2(valid_out) -> Terminator/1
  valid_in/1 -> cmac4/5(valid_in)
  Concat/1 -> acc_out/1
  Slice5/1 -> cmac2/3(acc_in)
  Slice4/1 -> cmac2/2(c+di)
  Slice3/1 -> cmac2/1(a+bi)
  Slice2/1 -> cmac1/3(acc_in)
  Slice1/1 -> cmac1/2(c+di)
  Slice/1 -> cmac1/1(a+bi)
  Constant2/1 -> cmac1/5(valid_in)

== system s_b4a4x32kf/sys0/xeng/window_delay/negedge ==
  in : Inport
  Delay : xbsIndex_r4/Delay  rst=off  infoeditControl=Selection of Reset will increase slice count due to use of real FFs and instead of SRLs  en=off  latency=1  reg_retiming=off  dbl_ovrd=off  block_type=delay
      settings: xl_area=[0, 0, 0, 0, 0, 0, 0]
  Inverter : xbsIndex_r4/Inverter  en=off  latency=0  dbl_ovrd=off  block_type=inv
      settings: xl_area=[0, 0, 0, 0, 0, 0, 0]
  edge_op : xbsIndex_r4/Logical  logical_function=AND  inputs=2  en=off  latency=0  precision=Full  arith_type=Unsigned  n_bits=8  bin_pt=2  align_bp=on  dbl_ovrd=off  block_type=logical
      settings: xl_area=[0, 0, 0, 0, 0, 0, 0]
  out : Outport
  wires:
  Delay/1 -> edge_op/2
  in/1 -> Delay/1, Inverter/1
  edge_op/1 -> out/1
  Inverter/1 -> edge_op/1

== system s_b4a4x32kf/sys0/xeng/window_delay/posedge3 ==
  in : Inport
  Delay : xbsIndex_r4/Delay  rst=off  infoeditControl=Selection of Reset will increase slice count due to use of real FFs and instead of SRLs  en=off  latency=1  reg_retiming=off  dbl_ovrd=off  block_type=delay
      settings: xl_area=[0, 0, 0, 0, 0, 0, 0]
  Inverter : xbsIndex_r4/Inverter  en=off  latency=0  dbl_ovrd=off  block_type=inv
      settings: xl_area=[0, 0, 0, 0, 0, 0, 0]
  edge_op : xbsIndex_r4/Logical  logical_function=NOR  inputs=2  en=off  latency=0  precision=Full  arith_type=Unsigned  n_bits=8  bin_pt=2  align_bp=on  dbl_ovrd=off  block_type=logical
      settings: xl_area=[0, 0, 0, 0, 0, 0, 0]
  out : Outport
  wires:
  Delay/1 -> edge_op/2
  in/1 -> Delay/1, Inverter/1
  edge_op/1 -> out/1
  Inverter/1 -> edge_op/1

== system s_b4a4x32kf/sys0/xeng/window_delay/sync_delay ==
  In : Inport
  Constant : xbsIndex_r4/Constant  const=1  gui_display_data_type=Fixed-point  arith_type=Unsigned  n_bits=BitWidth  bin_pt=0  preci_type=Single  exp_width=8  frac_width=24  explicit_period=on  period=1  equ=P=C  opselect=C  inp2=PCIN>>17  opr=+  inp1=P  carry=CIN  dbl_ovrd=off  block_type=constant
      settings: block_version=9.1.01
  Constant1 : xbsIndex_r4/Constant  const=0  gui_display_data_type=Fixed-point  arith_type=Unsigned  n_bits=BitWidth  bin_pt=0  preci_type=Single  exp_width=8  frac_width=24  explicit_period=on  period=1  equ=P=C  opselect=C  inp2=PCIN>>17  opr=+  inp1=P  carry=CIN  dbl_ovrd=off  block_type=constant
      settings: block_version=9.1.01
  Constant2 : xbsIndex_r4/Constant  const=DelayLen  gui_display_data_type=Fixed-point  arith_type=Unsigned  n_bits=BitWidth  bin_pt=0  preci_type=Single  exp_width=8  frac_width=24  explicit_period=on  period=1  equ=P=C  opselect=C  inp2=PCIN>>17  opr=+  inp1=P  carry=CIN  dbl_ovrd=off  block_type=constant
      settings: block_version=9.1.01
  Constant3 : xbsIndex_r4/Constant  const=UseCounter  gui_display_data_type=Fixed-point  arith_type=Unsigned  n_bits=1  bin_pt=0  preci_type=Single  exp_width=8  frac_width=24  explicit_period=on  period=1  equ=P=C  opselect=C  inp2=PCIN>>17  opr=+  inp1=P  carry=CIN  dbl_ovrd=off  block_type=constant
      settings: block_version=9.1.01
  Counter : xbsIndex_r4/Counter  cnt_type=Free Running  cnt_to=Inf  operation=Down  start_count=0  cnt_by_val=1  arith_type=Unsigned  n_bits=BitWidth  bin_pt=0  load_pin=on  rst=off  en=on  explicit_period=on  period=1  use_behavioral_HDL=off  implementation=Fabric  use_rpm=on  dbl_ovrd=off  block_type=counter
      settings: xl_area=[0, 0, 0, 0, 0, 0, 0]  block_version=9.1.01
  Logical : xbsIndex_r4/Logical  logical_function=OR  inputs=2  en=off  latency=0  precision=Full  arith_type=Unsigned  n_bits=8  bin_pt=2  align_bp=on  dbl_ovrd=off  block_type=logical
      settings: xl_area=[0, 0, 0, 0, 0, 0, 0]  block_version=9.1.01
  Mux : xbsIndex_r4/Mux  inputs=2  en=off  latency=0  precision=Full  arith_type="Signed  (2's comp)"  n_bits=8  bin_pt=2  quantization=Truncate  overflow=Wrap  dbl_ovrd=off  block_type=mux
      settings: xl_area=[0, 0, 0, 0, 0, 0, 0]  block_version=9.1.01
  Relational : xbsIndex_r4/Relational  mode=a=b  op_type=Bool  en=off  latency=0  dbl_ovrd=off  block_type=relational
      settings: xl_area=[0, 0, 0, 0, 0, 0, 0]  block_version=9.1.01
  Relational1 : xbsIndex_r4/Relational  mode=a!=b  op_type=Bool  en=off  latency=0  dbl_ovrd=off  block_type=relational
      settings: xl_area=[0, 0, 0, 0, 0, 0, 0]  block_version=9.1.01
  warn period Logical0 : xbsReplacements_r4/Warning  period=1
  warn period Relational10 : xbsReplacements_r4/Warning  period=1
  Out : Outport
  wires:
  Mux/1 -> Out/1
  Constant3/1 -> Mux/1
  Relational/1 -> Mux/3
  Relational1/1 -> Logical/2
  Logical/1 -> Counter/3
  In/1 -> Mux/2, Logical/1, Counter/1
  Constant2/1 -> Counter/2
  Constant/1 -> Relational/1
  Constant1/1 -> Relational1/2
  Counter/1 -> Relational/2, Relational1/1

== system s_b4a4x32kf/sys0/xeng/window_delay/sync_delay1 ==
  In : Inport
  Constant : xbsIndex_r4/Constant  const=1  gui_display_data_type=Fixed-point  arith_type=Unsigned  n_bits=BitWidth  bin_pt=0  preci_type=Single  exp_width=8  frac_width=24  explicit_period=on  period=1  equ=P=C  opselect=C  inp2=PCIN>>17  opr=+  inp1=P  carry=CIN  dbl_ovrd=off  block_type=constant
      settings: block_version=9.1.01
  Constant1 : xbsIndex_r4/Constant  const=0  gui_display_data_type=Fixed-point  arith_type=Unsigned  n_bits=BitWidth  bin_pt=0  preci_type=Single  exp_width=8  frac_width=24  explicit_period=on  period=1  equ=P=C  opselect=C  inp2=PCIN>>17  opr=+  inp1=P  carry=CIN  dbl_ovrd=off  block_type=constant
      settings: block_version=9.1.01
  Constant2 : xbsIndex_r4/Constant  const=DelayLen  gui_display_data_type=Fixed-point  arith_type=Unsigned  n_bits=BitWidth  bin_pt=0  preci_type=Single  exp_width=8  frac_width=24  explicit_period=on  period=1  equ=P=C  opselect=C  inp2=PCIN>>17  opr=+  inp1=P  carry=CIN  dbl_ovrd=off  block_type=constant
      settings: block_version=9.1.01
  Constant3 : xbsIndex_r4/Constant  const=UseCounter  gui_display_data_type=Fixed-point  arith_type=Unsigned  n_bits=1  bin_pt=0  preci_type=Single  exp_width=8  frac_width=24  explicit_period=on  period=1  equ=P=C  opselect=C  inp2=PCIN>>17  opr=+  inp1=P  carry=CIN  dbl_ovrd=off  block_type=constant
      settings: block_version=9.1.01
  Counter : xbsIndex_r4/Counter  cnt_type=Free Running  cnt_to=Inf  operation=Down  start_count=0  cnt_by_val=1  arith_type=Unsigned  n_bits=BitWidth  bin_pt=0  load_pin=on  rst=off  en=on  explicit_period=on  period=1  use_behavioral_HDL=off  implementation=Fabric  use_rpm=on  dbl_ovrd=off  block_type=counter
      settings: xl_area=[0, 0, 0, 0, 0, 0, 0]  block_version=9.1.01
  Logical : xbsIndex_r4/Logical  logical_function=OR  inputs=2  en=off  latency=0  precision=Full  arith_type=Unsigned  n_bits=8  bin_pt=2  align_bp=on  dbl_ovrd=off  block_type=logical
      settings: xl_area=[0, 0, 0, 0, 0, 0, 0]  block_version=9.1.01
  Mux : xbsIndex_r4/Mux  inputs=2  en=off  latency=0  precision=Full  arith_type="Signed  (2's comp)"  n_bits=8  bin_pt=2  quantization=Truncate  overflow=Wrap  dbl_ovrd=off  block_type=mux
      settings: xl_area=[0, 0, 0, 0, 0, 0, 0]  block_version=9.1.01
  Relational : xbsIndex_r4/Relational  mode=a=b  op_type=Bool  en=off  latency=0  dbl_ovrd=off  block_type=relational
      settings: xl_area=[0, 0, 0, 0, 0, 0, 0]  block_version=9.1.01
  Relational1 : xbsIndex_r4/Relational  mode=a!=b  op_type=Bool  en=off  latency=0  dbl_ovrd=off  block_type=relational
      settings: xl_area=[0, 0, 0, 0, 0, 0, 0]  block_version=9.1.01
  warn period Logical0 : xbsReplacements_r4/Warning  period=1
  warn period Relational10 : xbsReplacements_r4/Warning  period=1
  Out : Outport
  wires:
  Mux/1 -> Out/1
  Constant3/1 -> Mux/1
  Relational/1 -> Mux/3
  Relational1/1 -> Logical/2
  Logical/1 -> Counter/3
  In/1 -> Mux/2, Logical/1, Counter/1
  Constant2/1 -> Counter/2
  Constant/1 -> Relational/1
  Constant1/1 -> Relational1/2
  Counter/1 -> Relational/2, Relational1/1
